simulink model "dcMotorControlSim_HexaMotor"  (R2026a)
settings: Solver=ode15s  StopTime=10
PreLoadFcn:
  | dcMotorControlInit_HexaMotor
values from neighbouring files (symbols this model uses):
  hexaMotor = hexaMotorParams()    [dcMotorControlInit_HexaMotor.m]
  sampleTime = 0.01    [dcMotorControlInit.m]    (also in dcMotorControlInit_HexaMotor.m = hexaMotor.sampleTime)
libraries: fl_lib x15, nesl_utility x9, ee_lib x4, slpidlib x1, eeGeneralControl x1, sdl_lib x1
Description:
  | DC Motor Control Simulation
settings Model: Creator=ControlLab  LastModifiedBy=arkad
settings SimscapeCC: SimscapeNominalValues="[{\"value\":\"1\",\"unit\":\"A\"},{\"value\":\"1\",\"unit\":\"bar\"},{\"value\":\"1\",\"unit\":\"cm^2\"},{\"value\":\"1\",\"unit\":\"cm^3/s\"},{\"value\":\"1\",\"unit\":\"kJ/kg\"},{\"value\":\"1\",\"unit\":\"kW\"},{\"value\":\"1\",\"unit\":\"l\"},{\"value\":\"1\",\"unit\":\"N\"},{\"value\":\"1\",\"unit\":\"N*m\"},{\"value\":\"1\",\"unit\":\"V\"}]"  SimscapeLogType=none  SimscapeLogDataHistory=5000.0

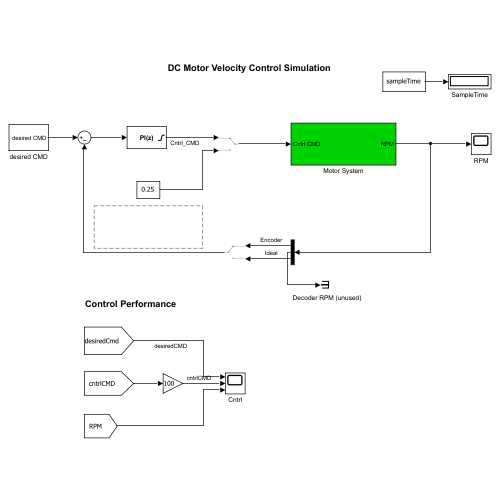
[thumbnail: Simulink's stored preview of the top-level diagram]
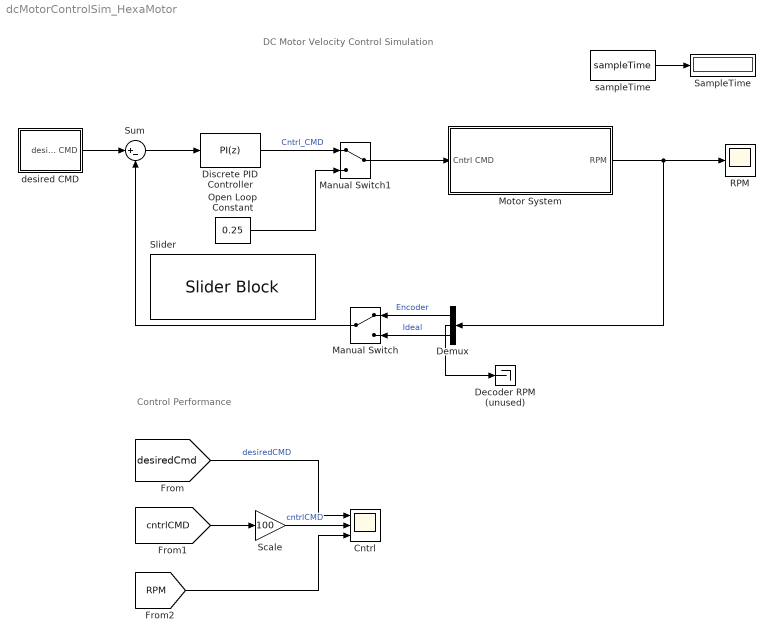
== system dcMotorControlSim_HexaMotor ==
  note: Control Performance
  note: DC Motor Velocity Control Simulation
  Cntrl : Scope  NumInputPorts=3
      settings: Title="Control  Performance"  ActiveDisplayYMinimum=-125.62995  ActiveDisplayYMaximum=130.66958  DataLoggingVariableName=ScopeData2
  Decoder RPM (unused) : Terminator
  Demux : Demux  Outputs=3
  Discrete PID Controller : slpidlib/PID Controller  Controller=PI  Form=Parallel  TimeDomain=Discrete-time  UseExternalTs=off  SampleTime=sampleTime  IntegratorMethod=Forward Euler  FilterMethod=Forward Euler  ControllerParametersSource=internal  P=hexaMotor.Kp_duty  I=hexaMotor.Ki_duty  UseKiTs=off  D=0.0001  UseExternalDerivativeSource=off  N=0  UseFilter=off  TunerSelectOption=Transfer Function Based (PID Tuner App)  InitialConditionSource=internal  InitialConditionForIntegrator=0  InitialConditionForFilter=0  DifferentiatorICPrevScaledInput=0  ExternalReset=none  TrackingMode=off  Kt=1  LimitOutput=on  SatLimitsSource=internal  UpperSaturationLimit=1  LowerSaturationLimit=-1  LinearizeAsGain=on  AntiWindupMode=back-calculation  Kb=1  LimitIntegrator=off  UpperIntegratorSaturationLimit=inf  LowerIntegratorSaturationLimit=-inf  POutMin=[]  POutMax=[]  IOutMin=[]  IOutMax=[]  DOutMin=[]  DOutMax=[]  NOutMin=[]  NOutMax=[]  SumOutMin=[]  SumOutMax=[]  SaturationOutMin=[]  SaturationOutMax=[]  PParamMin=[]  PParamMax=[]  IParamMin=[]  IParamMax=[]  DParamMin=[]  DParamMax=[]  NParamMin=[]  NParamMax=[]  KbParamMin=[]  KbParamMax=[]  KtParamMin=[]  KtParamMax=[]  KbOutMin=[]  KbOutMax=[]  KtOutMin=[]  KtOutMax=[]  IntegratorOutMin=[]  IntegratorOutMax=[]  FilterOutMin=[]  FilterOutMax=[]  SumI1OutMin=[]  SumI1OutMax=[]  SumI2OutMin=[]  SumI2OutMax=[]  SumI3OutMin=[]  SumI3OutMax=[]  SumI4OutMin=[]  SumI4OutMax=[]  SumDOutMin=[]  SumDOutMax=[]  DifferentiatorOutMin=[]  DifferentiatorOutMax=[]  FilterDiffOutCoefMin=[]  FilterDiffOutCoefMax=[]  ReciprocalOutMin=[]  ReciprocalOutMax=[]  SumDenOutMin=[]  SumDenOutMax=[]  SumNumOutMin=[]  SumNumOutMax=[]  DivideOutMin=[]  DivideOutMax=[]  UdiffTsProdOutMin=[]  UdiffTsProdOutMax=[]  NTsProdOutMin=[]  NTsProdOutMax=[]  UintegralTsProdOutMin=[]  UintegralTsProdOutMax=[]  UngainTsProdOutMin=[]  UngainTsProdOutMax=[]  ClampingZeroOutDataTypeStr=Inherit: Inherit via back propagation  ClampingZeroOutMin=[]  ClampingZeroOutMax=[]  FilterDenConstantOutDataTypeStr=Inherit: Inherit via back propagation  FilterDenConstantOutMin=[]  FilterDenConstantOutMax=[]  PCopyOutDataTypeStr=Inherit: Inherit via back propagation  PCopyOutMin=[]  PCopyOutMax=[]  NCopyOutDataTypeStr=Inherit: Inherit via back propagation  NCopyOutMin=[]  NCopyOutMax=[]  IntegratorContinuousStateAttributes=''  IntegratorStateMustResolveToSignalObject=off  IntegratorRTWStateStorageClass=Auto  FilterContinuousStateAttributes=''  FilterStateMustResolveToSignalObject=off  FilterRTWStateStorageClass=Auto  ParallelPVariant=InternalParameters  IdealPVariant=Disabled  IVariant=InternalParameters  DVariant=Disabled  IntegratorVariant=Discrete  SatVariant=Enabled  AWVariant=BackCalculation  PCopyVariant=Disabled  TRVariant=Disabled  FdbkBlocksVariant=Forward  IdealPFdbkVariant=Disabled  SatFdbkVariant=Disabled  DerivativeFilterVariant=Disabled  NVariant=Disabled  NCopyVariant=Disabled_SignalSpec  FilterICVariant=Disabled  IntegratorICVariant=InternalICs  ExternalResetVariant=Disabled  TRSumVariant=Passthrough  SumFdbkVariant=Disabled  SumVariant=Sum_PI  TsampFilterVariant=InternalTs  TsampNgainVariant=Passthrough  TsampIntegralVariant=Disabled_SignalSpec  ExternalSaturationOutDataTypeStr=Inherit: Same as second input  DerivativeSourceVariant=Disabled  PreIntVariant=InternalPreInt
  Manual Switch : ManualSwitch
  Manual Switch1 : ManualSwitch
  Motor System : Subsystem
  Open Loop Constant : Constant  Value=0.25  SampleTime=sampleTime
  RPM : Scope
      settings: ActiveDisplayYMinimum=-130.81519  ActiveDisplayYMaximum=201.86786  DataLoggingVariableName=RPM
  SampleTime : Display
  Scale : Gain  Gain=100
  Slider : SliderBlock  ScaleMin=-1  ScaleMax=1
  Sum : Sum  Inputs=|+-
  desired CMD : Subsystem
  sampleTime : Constant  Value=sampleTime  SampleTime=sampleTime
  wires:
  Open Loop Constant/1 -> Manual Switch1/2
  Manual Switch1/1 -> Motor System/1(Cntrl CMD)
  Discrete PID Controller/1 -> Manual Switch1/1  "Cntrl_CMD"
  Sum/1 -> Discrete PID Controller/1
  Demux/2 -> Manual Switch/2  "Ideal"
  desired CMD/1(desired CMD) -> Sum/1
  Motor System/1(RPM) -> Demux/1, RPM/1
  Manual Switch/1 -> Sum/2
  Demux/1 -> Manual Switch/1  "Encoder"
  sampleTime/1 -> SampleTime/1
  [desiredCmd] -> Cntrl/1  "desiredCMD"
  [cntrlCMD] -> Scale/1
  Scale/1 -> Cntrl/2  "cntrlCMD"
  [RPM] -> Cntrl/3
  Demux/3 -> Decoder RPM (unused)/1

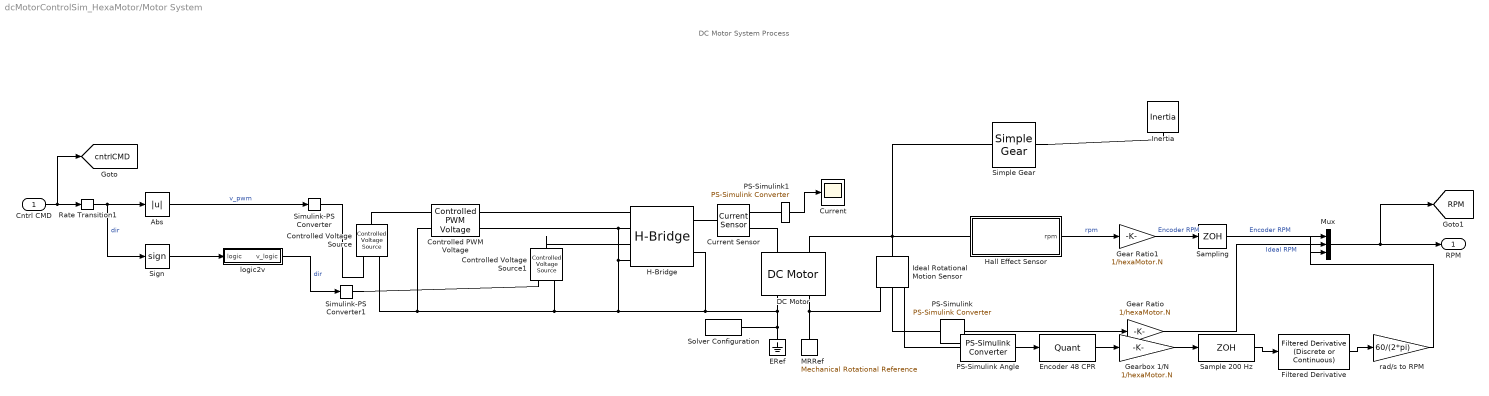
== system dcMotorControlSim_HexaMotor/Motor System ==
  note: DC Motor System Process
  Cntrl CMD : Inport
  Abs : Abs  SaturateOnIntegerOverflow=off
  Controlled PWM Voltage : ee_lib/Integrated Circuits/Controlled PWM Voltage  F=512 Hz  TD=0 s  pulse_width_offset=0 s  pulse_min=0 s  pwm_or_av=2  event_type=1  sample_time=5e-6 s  Vmin=0 V  Vmax=1 V  Vm=5 V  u_min=0  u_max=1
  Controlled Voltage Source : fl_lib/Electrical/Electrical Sources/Controlled Voltage Source
  Controlled Voltage Source1 : fl_lib/Electrical/Electrical Sources/Controlled Voltage Source
  Current : Scope
      settings: TimeSpan=10  ActiveDisplayYMinimum=-0.5  ActiveDisplayYMaximum=2  DataLoggingVariableName=RPM
  Current Sensor : fl_lib/Electrical/Electrical Sensors/Current Sensor
  DC Motor : ee_lib/Electromechanical/Brushed Motors/DC Motor  field_option=ee.enum.field_option.pm  Rf=100 Ohm  Lf=1 H  Laf=0.15 H  If0=0 A  parameterization=ee.enum.dcparam_option.circuit_param  Ra=hexaMotor.Ra Ohm  La=hexaMotor.La H  emf_or_torque=ee.enum.emf_or_torque.kv  Kv=hexaMotor.K V/(rad/s)  Ki=6.876e-04 N*m/A  T_stall=0.001274 N*m  w_max=33000 rpm  w_rated=17000 rpm  P_rated=1.1 W  V_rated=12 V  lam_param=ee.enum.lam_param.damping  i_noload=0.054 A  V_i_noload=2.5 V  J=hexaMotor.Jmotor kg*m^2  lam=hexaMotor.damping N*m/(rad/s)  speed0=0 rpm  alpha=3.93e-3 1/K  Tmeas=25 degC  thermal_mass=100 J/K  initial_temperature=25 degC
  ERef : fl_lib/Electrical/Electrical Elements/Electrical Reference
  Encoder 48 CPR : Quantizer  QuantizationInterval=2*pi/hexaMotor.encCPR
  Filtered Derivative : eeGeneralControl/Filtered Derivative (Discrete or Continuous)  K=1  T=0.05  B=inf  A=-inf  minRatio=10  init_option=Inherited from block input  x0=0  Ts=-1
      settings: LibrarySourceBlock=|
      | ee_sl_lib/General Control/Filtered Derivative
      | (Discrete or Continuous)
  Gear Ratio : Gain  Gain=1/hexaMotor.N
  Gear Ratio1 : Gain  Gain=1/hexaMotor.N
  Gearbox 1/N : Gain  Gain=1/hexaMotor.N
  H-Bridge : ee_lib/Semiconductors & Converters/Converters/H-Bridge  pwm_or_av=2  discontinuous=0  freewheeling_mode=1  Rload=hexaMotor.Ra + 0.1 Ohm  Lload=1e-5 H  F=4 kHz  supply_ports=ee.enum.supply_ports.hidesupply  regenerative_braking_mode=2  Venable=2.5 V  Vmax=5 V  Vreverse=2.5 V  Vbrake=2.5 V  Vm=hexaMotor.Vsupply V  Ron=0.1 Ohm  Don=0.1 Ohm  Goff=1e-6 S  Tmeas=298.15 K  Ron2=0.1 Ohm  Don2=0.05 Ohm  Tmeas2=398.15 K  thermal_mass=100 J/K  initial_temperature=298.15 K
  Hall Effect Sensor : Subsystem
  Ideal Rotational Motion Sensor : fl_lib/Mechanical/Mechanical Sensors/Ideal Rotational Motion Sensor  reference=foundation.enum.MeasurementReference.difference  acceleration_port=false  velocity_port=true  position_port=true  wrap_angle=simscape.enum.onoff.off  offset=0 deg
  Inertia : fl_lib/Mechanical/Rotational Elements/Inertia  inertia=hexaMotor.Jload kg*m^2  num_ports=foundation.enum.numPorts2.one  w_specify=on  w_priority=None  w=0 rad/s  w_nominal_specify=off  w_nominal_value=1  w_nominal_unit=rad/s  t_specify=off  t_priority=High  t=0 N*m  t_nominal_specify=off  t_nominal_value=1  t_nominal_unit=N*m
  MRRef : fl_lib/Mechanical/Rotational Elements/Mechanical Rotational Reference
  Mux : Mux  Inputs=3
  PS-Simulink : nesl_utility/PS-Simulink Converter  PhysicalDomain=network_engine_domain  SubClassName=ps_output  LeftPortType=input  RightPortType=output  PseudoPeriodic=off  Frequencies=[]  VectorFormat=1-D array  Unit=rpm  AffineConversion=off
  PS-Simulink Angle : nesl_utility/PS-Simulink Converter  PhysicalDomain=network_engine_domain  SubClassName=ps_output  LeftPortType=input  RightPortType=output  PseudoPeriodic=off  Frequencies=[]  VectorFormat=1-D array  Unit=rad  AffineConversion=off
  PS-Simulink1 : nesl_utility/PS-Simulink Converter  PhysicalDomain=network_engine_domain  SubClassName=ps_output  LeftPortType=input  RightPortType=output  PseudoPeriodic=off  Frequencies=[]  VectorFormat=1-D array  Unit=A  AffineConversion=off
  Rate Transition1 : RateTransition
  Sample 200 Hz : ZeroOrderHold  SampleTime=sampleTime
  Sampling : ZeroOrderHold  SampleTime=sampleTime
  Sign : Signum
  Simple Gear : sdl_lib/Gears/Simple Gear  ratio=hexaMotor.N  rotation_direction=3-2*(1)  friction_model=sdl.enum.gear_efficiencies_load.constant  T_noload=0.1 N*m  T_nom=5 N*m  efficiency_nom=0.8  efficiency=hexaMotor.gearEff  temperature_TLU=[280, 300, 320] K  load_TLU=[1, 5, 10] N*m  efficiency_TLU=[.95, .9, .85]  efficiency_TLU2=[.85, .8, .75; .95, .9, .85; .85, .8, .7]  w_thr=0.01 rad/s  pwr_thr=0.1 W  enable_backlash=false  hardstop_model=simscape.enum.hardstop.smooth  backlash_distance=1e-3 mm  r_base=0.1 m  transition=1e-4 mm  backlash_stiffness=1e6 N/m  backlash_damping=1e3 N*s/m  coeff_rest=0.7  v_tol=0.001 m/s  f_tol=0 N  tau=0.1 s  mu_visc=[0, 0] N*m/(rad/s)  thermal_mass=50 J/K  temperature_specify=off  temperature_priority=High  temperature=300 K  temperature_nominal_specify=off  temperature_nominal_value=1  temperature_nominal_unit=K  x_backlash_specify=off  x_backlash_priority=None  x_backlash=0 mm  x_backlash_nominal_specify=off  x_backlash_nominal_value=1  x_backlash_nominal_unit=mm  f_hardstop_specify=off  f_hardstop_priority=None  f_hardstop=0 N  f_hardstop_nominal_specify=off  f_hardstop_nominal_value=1  f_hardstop_nominal_unit=N  v_backlash_specify=off  v_backlash_priority=None  v_backlash=0 m/s  v_backlash_nominal_specify=off  v_backlash_nominal_value=1  v_backlash_nominal_unit=m/s
  Simulink-PS Converter : nesl_utility/Simulink-PS Converter  PhysicalDomain=network_engine_domain  SubClassName=ps_input  LeftPortType=input  RightPortType=output  PseudoPeriodic=off  Frequencies=[]  NoiseDistribution=none  NoiseParameters=[]  Unit=1  AffineConversion=off  FilteringAndDerivatives=provide  SimscapeFilterOrder=1  InputFilterTimeConstant=0.001  UdotUserProvided=0
  Simulink-PS Converter1 : nesl_utility/Simulink-PS Converter  PhysicalDomain=network_engine_domain  SubClassName=ps_input  LeftPortType=input  RightPortType=output  PseudoPeriodic=off  Frequencies=[]  NoiseDistribution=none  NoiseParameters=[]  Unit=1  AffineConversion=off  FilteringAndDerivatives=provide  SimscapeFilterOrder=1  InputFilterTimeConstant=0.001  UdotUserProvided=0
  Solver Configuration : nesl_utility/Solver Configuration  PhysicalDomain=network_engine_domain  SubClassName=solver  LeftPortType=input  RightPortType=generic  Tones=[]  Harmonics=[]  SimulateNoise=off  Profile=off  UseLocalSampling=off  EnableSwitchedLinearOptims=on  FrequencyDomain=off  UseCCode=off  RelTol=0.001  AbsTol=1e-06  MinStep=1e-09  ToWorkspace=off  RevertToSquareIcSolve=off  NumHomotopyIterations=100  PhasorMode=off  PhasorModeNumHarmonics=1  ConsistencySolver=NEWTON_FTOL  CanonicalOrdering=UNORDERED  OptimizeIntermediates=UNOPTIMIZED  IndexReductionMethod=DerivativeReplacement  DoDC=off  ResidualTolerance=1e-9  ConsistencyTolSource=GLOBAL  ConsistencyAbsTol=0.001  ConsistencyRelTol=0.001  ConsistencyTolFactor=0.001  UseLocalSolver=off  LocalSolverChoice=NE_BACKWARD_EULER_ADVANCER  ResolveIndetEquations=on  FunctionEvalNumThread=1  LocalSolverSampleTime=5e-6  DoFixedCost=off  MaxNonlinIter=4  MaxModeIter=2  ComputeImpulses=off  ImpulseIterations=2  LinearAlgebra=auto  LinearAlgebraNumThread=0  EquationFormulation=NE_TIME_EF  DelaysMemoryBudget=1024  AutomaticFiltering=on  FilteringTimeConstant=0.001  PartitionStorageMethod=AS_NEEDED  PartitionMemoryBudget=1024  PartitionMethod=FAST  MultibodyUseLocalSolver=off  MultibodyLocalSolverChoice=ODE1  MultibodyLocalSolverSampleTime=0.001
  logic2v : Subsystem
  rad/s to RPM : Gain  Gain=60/(2*pi)
  RPM : Outport
  tag scope: RPM=global, cntrlCMD=global
  wires:
  logic2v/1(v_logic) -> Simulink-PS Converter1/1  "dir"
  PS-Simulink1/1 -> Current/1
  Hall Effect Sensor/1(rpm) -> Gear Ratio1/1  "rpm"
  Gear Ratio1/1 -> Sampling/1  "Encoder RPM"
  Gear Ratio/1 -> Mux/2  "Ideal RPM"
  PS-Simulink/1 -> Gear Ratio/1
  Mux/1 -> [RPM], RPM/1
  Cntrl CMD/1 -> [cntrlCMD], Rate Transition1/1
  Abs/1 -> Simulink-PS Converter/1  "v_pwm"
  Sign/1 -> logic2v/1(logic)
  Rate Transition1/1 -> Sign/1, Abs/1  "dir"
  PS-Simulink Angle/1 -> Encoder 48 CPR/1
  Encoder 48 CPR/1 -> Gearbox 1/N/1
  Gearbox 1/N/1 -> Sample 200 Hz/1
  Sample 200 Hz/1 -> Filtered Derivative/1
  Filtered Derivative/1 -> rad/s to RPM/1
  rad/s to RPM/1 -> Mux/1
  Sampling/1 -> Mux/3  "Encoder RPM"
  connections:
  Controlled Voltage Source/LConn1 -- Controlled PWM Voltage/LConn1
  Controlled Voltage Source/RConn2 -- Controlled PWM Voltage/LConn2 -- Controlled Voltage Source1/RConn2 -- H-Bridge/LConn2 -- Controlled PWM Voltage/RConn2 -- H-Bridge/LConn4 -- DC Motor/RConn1 -- Solver Configuration/RConn1 -- ERef/LConn1 -- H-Bridge/RConn2
  DC Motor/RConn2 -- MRRef/LConn1 -- Ideal Rotational Motion Sensor/RConn1
  H-Bridge/RConn1 -- Current Sensor/LConn1
  Current Sensor/RConn2 -- DC Motor/LConn1
  DC Motor/LConn2 -- Simple Gear/LConn1 -- Ideal Rotational Motion Sensor/LConn1 -- Hall Effect Sensor/LConn1
  H-Bridge/LConn1 -- Controlled PWM Voltage/RConn1
  Controlled Voltage Source1/LConn1 -- H-Bridge/LConn3
  Simulink-PS Converter/RConn1 -- Controlled Voltage Source/RConn1
  Current Sensor/RConn1 -- PS-Simulink1/LConn1
  Simulink-PS Converter1/RConn1 -- Controlled Voltage Source1/RConn1
  PS-Simulink/LConn1 -- Ideal Rotational Motion Sensor/RConn2
  Simple Gear/RConn1 -- Inertia/LConn1
  Ideal Rotational Motion Sensor/RConn3 -- PS-Simulink Angle/LConn1

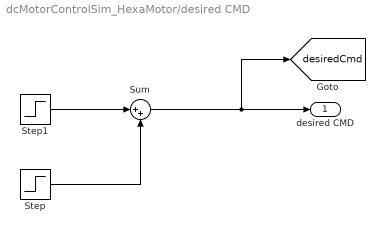
== system dcMotorControlSim_HexaMotor/desired CMD ==
  Step : Step  Time=7  FinalValue=-100  SampleTime=sampleTime
  Step1 : Step  FinalValue=100  SampleTime=sampleTime
  Sum : Sum  Inputs=|++
  desired CMD : Outport
  tag scope: desiredCmd=global
  wires:
  Step/1 -> Sum/2
  Step1/1 -> Sum/1
  Sum/1 -> [desiredCmd], desired CMD/1

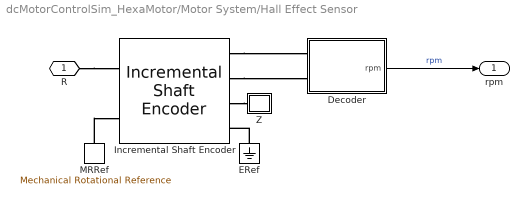
== system dcMotorControlSim_HexaMotor/Motor System/Hall Effect Sensor ==
  Decoder : Subsystem
  ERef : fl_lib/Electrical/Electrical Elements/Electrical Reference
  Incremental Shaft Encoder : ee_lib/Sensors & Transducers/Incremental Shaft Encoder  NPulse=hexaMotor.encPPR  Vm=5 V  angle0=-1 deg
  MRRef : fl_lib/Mechanical/Rotational Elements/Mechanical Rotational Reference
  Z : Subsystem
  R : PMIOPort  Side=Left
  rpm : Outport  VectorParamsAs1DForOutWhenUnconnected=off
  wires:
  Decoder/1(rpm) -> rpm/1  "rpm"
  connections:
  MRRef/LConn1 -- Incremental Shaft Encoder/LConn2
  R/RConn1 -- Incremental Shaft Encoder/LConn1
  ERef/LConn1 -- Incremental Shaft Encoder/RConn4
  Incremental Shaft Encoder/RConn3 -- Z/LConn1
  Incremental Shaft Encoder/RConn2 -- Decoder/LConn2
  Incremental Shaft Encoder/RConn1 -- Decoder/LConn1

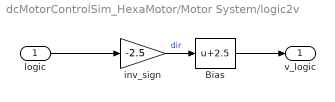
== system dcMotorControlSim_HexaMotor/Motor System/logic2v ==
  logic : Inport
  Bias : Bias  Bias=2.5  SaturateOnIntegerOverflow=off
  inv_sign : Gain  Gain=-2.5
  v_logic : Outport
  wires:
  inv_sign/1 -> Bias/1  "dir"
  logic/1 -> inv_sign/1
  Bias/1 -> v_logic/1

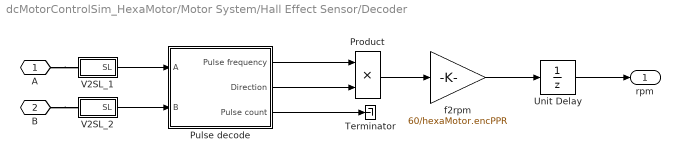
== system dcMotorControlSim_HexaMotor/Motor System/Hall Effect Sensor/Decoder ==
  Product : Product  RndMeth=Zero
  Pulse decode : Subsystem
  Terminator : Terminator
  Unit Delay : UnitDelay  SampleTime=sampleTime
  V2SL_1 : Subsystem
  V2SL_2 : Subsystem
  f2rpm : Gain  Gain=60/hexaMotor.encPPR
  A : PMIOPort  Side=Left
  B : PMIOPort  Port=2  Side=Left
  rpm : Outport  VectorParamsAs1DForOutWhenUnconnected=off
  wires:
  Product/1 -> f2rpm/1
  Pulse decode/2(Direction) -> Product/2
  Pulse decode/1(Pulse frequency) -> Product/1
  Pulse decode/3(Pulse count) -> Terminator/1
  V2SL_1/1(SL) -> Pulse decode/1(A)
  V2SL_2/1(SL) -> Pulse decode/2(B)
  f2rpm/1 -> Unit Delay/1
  Unit Delay/1 -> rpm/1
  connections:
  A/RConn1 -- V2SL_1/LConn1
  B/RConn1 -- V2SL_2/LConn1

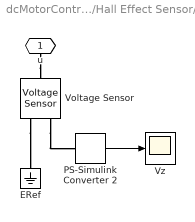
== system dcMotorControlSim_HexaMotor/Motor System/Hall Effect Sensor/Z ==
  ERef : fl_lib/Electrical/Electrical Elements/Electrical Reference
  PS-Simulink Converter 2 : nesl_utility/PS-Simulink Converter  PhysicalDomain=network_engine_domain  SubClassName=ps_output  LeftPortType=input  RightPortType=output  PseudoPeriodic=off  Frequencies=[]  VectorFormat=1-D array  Unit=V  AffineConversion=off
  Voltage Sensor : fl_lib/Electrical/Electrical Sensors/Voltage Sensor
  Vz : Scope
      settings: ActiveDisplayYMinimum=-1  ActiveDisplayYMaximum=6  DataLoggingVariableName=ScopeData6
  u : PMIOPort  Side=Left
  wires:
  PS-Simulink Converter 2/1 -> Vz/1
  connections:
  Voltage Sensor/RConn2 -- ERef/LConn1
  Voltage Sensor/RConn1 -- PS-Simulink Converter 2/LConn1
  u/RConn1 -- Voltage Sensor/LConn1

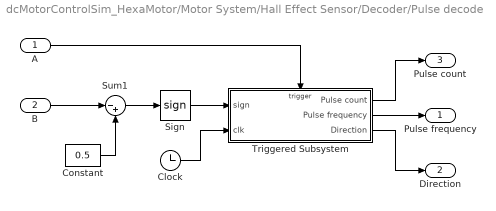
== system dcMotorControlSim_HexaMotor/Motor System/Hall Effect Sensor/Decoder/Pulse decode ==
  A : Inport
  B : Inport  Port=2
  Clock : Clock
  Constant : Constant  Value=0.5
  Sign : Signum
  Sum1 : Sum  Inputs=|-+
  Triggered Subsystem : Subsystem  TreatAsAtomicUnit=on
  Pulse frequency : Outport  VectorParamsAs1DForOutWhenUnconnected=off
  Direction : Outport  Port=2  VectorParamsAs1DForOutWhenUnconnected=off
  Pulse count : Outport  Port=3  VectorParamsAs1DForOutWhenUnconnected=off
  wires:
  Triggered Subsystem/3(Direction) -> Direction/1
  Triggered Subsystem/2(Pulse frequency) -> Pulse frequency/1
  Clock/1 -> Triggered Subsystem/2(clk)
  Triggered Subsystem/1(Pulse count) -> Pulse count/1
  A/1 -> Triggered Subsystem/Trigger
  Sign/1 -> Triggered Subsystem/1(sign)
  B/1 -> Sum1/1
  Sum1/1 -> Sign/1
  Constant/1 -> Sum1/2

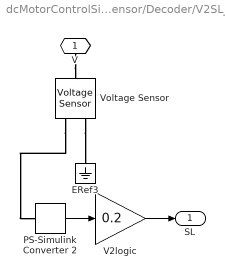
== system dcMotorControlSim_HexaMotor/Motor System/Hall Effect Sensor/Decoder/V2SL_1 ==
  ERef3 : fl_lib/Electrical/Electrical Elements/Electrical Reference
  PS-Simulink Converter 2 : nesl_utility/PS-Simulink Converter  PhysicalDomain=network_engine_domain  SubClassName=ps_output  LeftPortType=input  RightPortType=output  PseudoPeriodic=off  Frequencies=[]  VectorFormat=1-D array  Unit=V  AffineConversion=off
  V2logic : Gain  Gain=0.2
  Voltage Sensor : fl_lib/Electrical/Electrical Sensors/Voltage Sensor
  V : PMIOPort  Side=Left
  SL : Outport  VectorParamsAs1DForOutWhenUnconnected=off
  wires:
  PS-Simulink Converter 2/1 -> V2logic/1
  V2logic/1 -> SL/1
  connections:
  Voltage Sensor/RConn2 -- ERef3/LConn1
  V/RConn1 -- Voltage Sensor/LConn1
  Voltage Sensor/RConn1 -- PS-Simulink Converter 2/LConn1

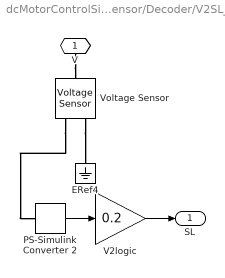
== system dcMotorControlSim_HexaMotor/Motor System/Hall Effect Sensor/Decoder/V2SL_2 ==
  ERef4 : fl_lib/Electrical/Electrical Elements/Electrical Reference
  PS-Simulink Converter 2 : nesl_utility/PS-Simulink Converter  PhysicalDomain=network_engine_domain  SubClassName=ps_output  LeftPortType=input  RightPortType=output  PseudoPeriodic=off  Frequencies=[]  VectorFormat=1-D array  Unit=V  AffineConversion=off
  V2logic : Gain  Gain=0.2
  Voltage Sensor : fl_lib/Electrical/Electrical Sensors/Voltage Sensor
  V : PMIOPort  Side=Left
  SL : Outport  VectorParamsAs1DForOutWhenUnconnected=off
  wires:
  V2logic/1 -> SL/1
  PS-Simulink Converter 2/1 -> V2logic/1
  connections:
  Voltage Sensor/RConn1 -- PS-Simulink Converter 2/LConn1
  V/RConn1 -- Voltage Sensor/LConn1
  Voltage Sensor/RConn2 -- ERef4/LConn1

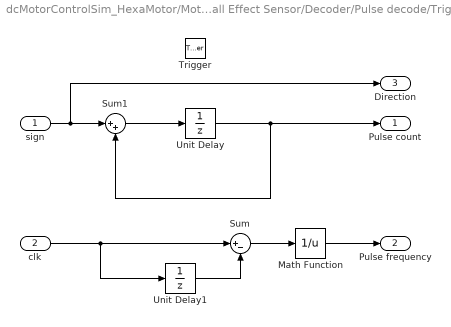
== system dcMotorControlSim_HexaMotor/Motor System/Hall Effect Sensor/Decoder/Pulse decode/Triggered Subsystem ==
  sign : Inport
  clk : Inport  Port=2
  Trigger : TriggerPort  VariantControl=Variant
  Math Function : Math  Operator=reciprocal  SignedPower=on
  Sum : Sum  Inputs=|+-
  Sum1 : Sum  Inputs=|++
  Unit Delay : UnitDelay  SampleTime=-1
  Unit Delay1 : UnitDelay  InitialCondition=-1e10  SampleTime=-1
  Pulse count : Outport  InitialOutput=0  VectorParamsAs1DForOutWhenUnconnected=off
  Pulse frequency : Outport  Port=2  VectorParamsAs1DForOutWhenUnconnected=off
  Direction : Outport  Port=3  InitialOutput=0  VectorParamsAs1DForOutWhenUnconnected=off
  wires:
  Math Function/1 -> Pulse frequency/1
  Sum/1 -> Math Function/1
  Unit Delay1/1 -> Sum/2
  clk/1 -> Sum/1, Unit Delay1/1
  Unit Delay/1 -> Sum1/2, Pulse count/1
  sign/1 -> Direction/1, Sum1/1
  Sum1/1 -> Unit Delay/1
